simulink model "classic_dtc_winder_clean"  (R2026a)
settings: Solver=VariableStepAuto  StopTime=Tsim  MaxStep=1e-6
undefined symbols (not defined in the file): B, C_web, draw_max, draw_takeup, F0, F_ref, F_slack, ff_full, ff_on, filt_on, Fmax, h, H0, HB_lambda, HB_torque, Jc, Jm, K_web, Ki_F, Ki_speed, Kp_F, Kp_speed, lambda_ref, p, r0, rc, rho, rmax, Rs, Rs_factor, T_ramp, t_rev, tau_F, Tmax, Ts_dtc, v_line_set, Vdc, w, w_max, w_min, w_ref, web_w, winder_mode_set
libraries: nesl_utility x13, fl_lib x10, ee_lib x5, slpidlib x2
settings Model: Creator=kunal  LastModifiedBy=kunal
settings SimscapeCC: SimscapeLogType=none

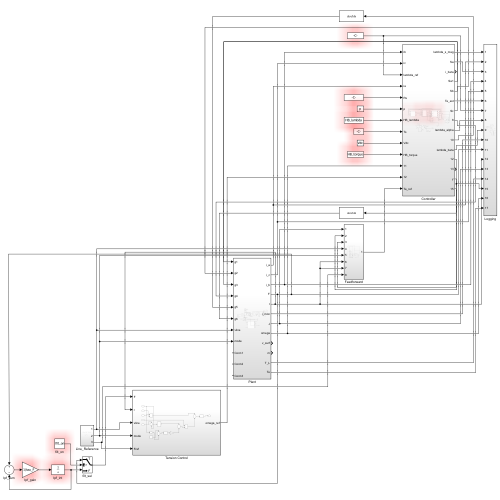
[thumbnail: Simulink's stored preview of the top-level diagram]
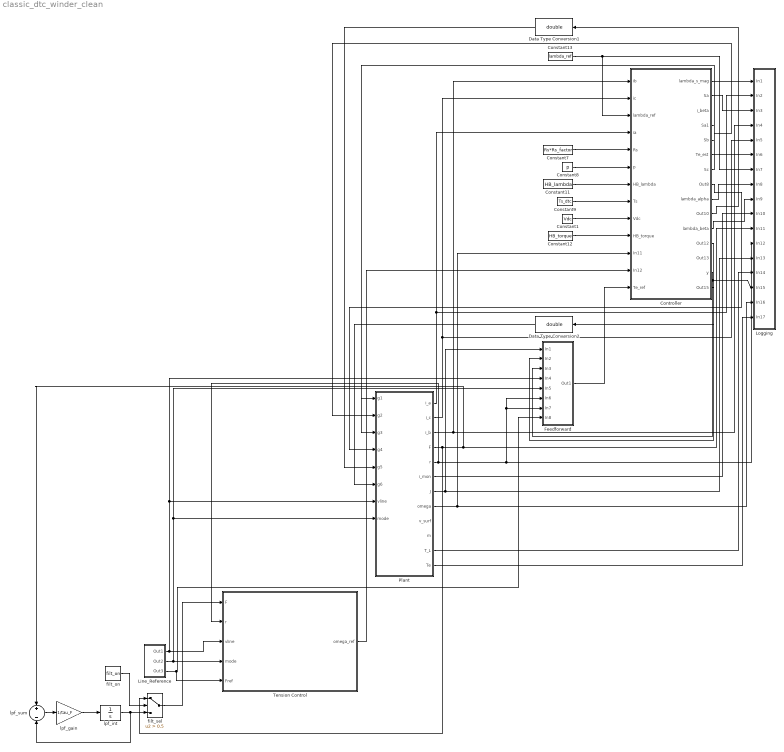
== system classic_dtc_winder_clean ==
  Constant1 : Constant  Value=Vdc
  Constant11 : Constant  Value=HB_lambda
  Constant12 : Constant  Value=HB_torque
  Constant13 : Constant  Value=lambda_ref
  Constant7 : Constant  Value=Rs*Rs_factor
  Constant8 : Constant  Value=p
  Constant9 : Constant  Value=Ts_dtc
  Controller : Subsystem
  Data Type Conversion1 : DataTypeConversion  OutDataTypeStr=double  SaturateOnIntegerOverflow=off  RndMeth=Floor
  Data Type Conversion2 : DataTypeConversion  OutDataTypeStr=double  SaturateOnIntegerOverflow=off  RndMeth=Floor
  Feedforward : Subsystem
  Line_Reference : Subsystem
  Logging : Subsystem
  Plant : Subsystem
  Tension Control : Subsystem
  filt_on : Constant  Value=filt_on
  filt_sel : Switch  Criteria=u2 > Threshold  Threshold=0.5  SaturateOnIntegerOverflow=off  InputSameDT=off
  lpf_gain : Gain  Gain=1/tau_F
  lpf_int : Integrator  InitialCondition=F0
  lpf_sum : Sum  Inputs=+-
  wires:
  lpf_sum/1 -> lpf_gain/1
  filt_on/1 -> filt_sel/2
  lpf_gain/1 -> lpf_int/1
  filt_sel/1 -> Tension Control/1(F)
  lpf_int/1 -> lpf_sum/2, filt_sel/3
  Line_Reference/3(Out3) -> Feedforward/8(In8), Tension Control/5(Fref)
  Line_Reference/1(Out1) -> Feedforward/4(In4), Plant/7(vline), Tension Control/3(vline)
  Line_Reference/2(Out2) -> Feedforward/5(In5), Plant/8(mode), Tension Control/4(mode)
  Plant/6(i_mon) -> Logging/10(In10)
  Plant/2(i_c) -> Logging/5(In5), Controller/2(ic)
  Tension Control/1(omega_ref) -> Controller/12(In12)
  Controller/1(lambda_s_mag) -> Logging/1(In1)
  Plant/1(i_a) -> Logging/2(In2), Controller/4(ia)
  Plant/11(T_L) -> Logging/14(In14)
  Plant/7(J) -> Logging/13(In13), Feedforward/1(In1)
  Plant/3(i_b) -> Controller/1(ib), Logging/4(In4)
  Plant/12(Te) -> Logging/17(In17)
  Plant/8(omega) -> Logging/16(In16), Controller/11(In11)
  Plant/4(F) -> lpf_sum/1, Logging/11(In11), filt_sel/1
  Plant/5(r) -> Feedforward/7(In7), Feedforward/6(In6), Logging/12(In12), Tension Control/2(r)
  Constant8/1 -> Controller/6(p)
  Data Type Conversion1/1 -> Plant/5(g5)
  Data Type Conversion2/1 -> Plant/6(g6)
  Constant11/1 -> Controller/7(HB_lambda)
  Constant13/1 -> Logging/7(In7), Controller/3(lambda_ref)
  Constant9/1 -> Controller/8(Ts)
  Constant7/1 -> Controller/5(Rs)
  Controller/11(lambda_beta) -> Logging/9(In9)
  Constant12/1 -> Controller/10(HB_torque)
  Constant1/1 -> Controller/9(Vdc)
  Feedforward/1(Out1) -> Controller/13(Te_ref)
  Controller/2(Sa) -> Logging/3(In3)
  Controller/4(Sa1) -> Plant/1(g1)
  Controller/5(Sb) -> Plant/2(g2)
  Controller/6(Te_est) -> Logging/6(In6)
  Controller/7(Sc) -> Plant/3(g3)
  Controller/8(Out8) -> Plant/4(g4)
  Controller/9(lambda_alpha) -> Logging/8(In8)
  Controller/10(Out10) -> Data Type Conversion1/1
  Controller/12(Out12) -> Data Type Conversion2/1
  Controller/14(y) -> Feedforward/3(In3), Logging/15(In15)
  Controller/15(Out15) -> Feedforward/2(In2)

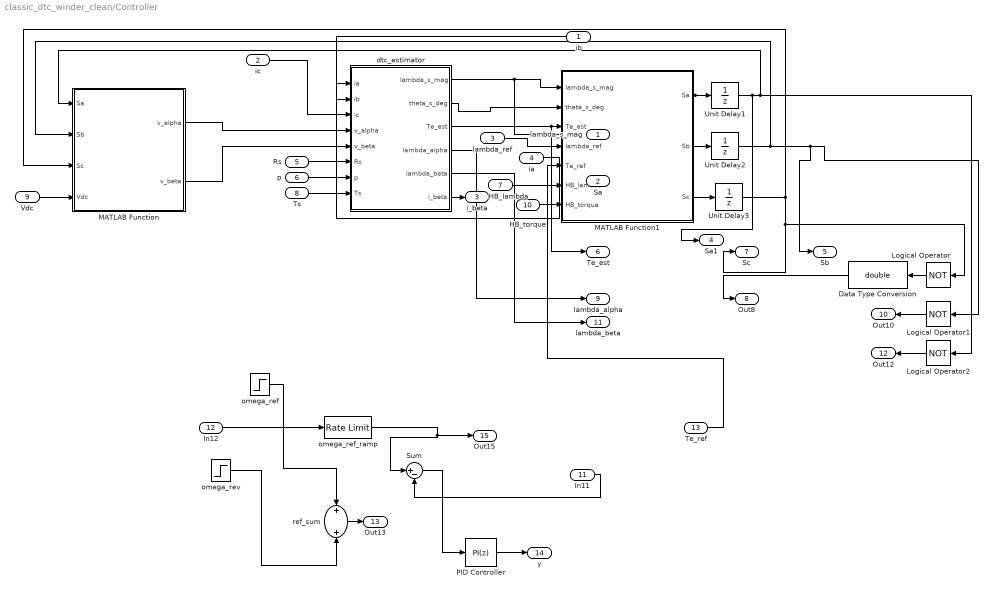
== system classic_dtc_winder_clean/Controller ==
  ib : Inport
  ic : Inport  Port=2
  lambda_ref : Inport  Port=3
  ia : Inport  Port=4
  Rs : Inport  Port=5
  p : Inport  Port=6
  HB_lambda : Inport  Port=7
  Ts : Inport  Port=8
  Vdc : Inport  Port=9
  HB_torque : Inport  Port=10
  In11 : Inport  Port=11
  In12 : Inport  Port=12
  Te_ref : Inport  Port=13
  Data Type Conversion : DataTypeConversion  OutDataTypeStr=double  SaturateOnIntegerOverflow=off  RndMeth=Floor
  Logical Operator : Logic  Operator=NOT  AllPortsSameDT=off  OutDataTypeStr=boolean
  Logical Operator1 : Logic  Operator=NOT  AllPortsSameDT=off  OutDataTypeStr=boolean
  Logical Operator2 : Logic  Operator=NOT  AllPortsSameDT=off  OutDataTypeStr=boolean
  MATLAB Function : MATLAB Function  TreatAsAtomicUnit=on  SystemSampleTime=Ts_dtc
  MATLAB Function1 : MATLAB Function  TreatAsAtomicUnit=on  SystemSampleTime=Ts_dtc
  PID Controller : slpidlib/PID Controller  Controller=PI  Form=Parallel  TimeDomain=Discrete-time  UseExternalTs=off  SampleTime=Ts_dtc  IntegratorMethod=Forward Euler  FilterMethod=Forward Euler  ControllerParametersSource=internal  P=Kp_speed  I=Ki_speed  UseKiTs=off  D=0  UseExternalDerivativeSource=off  N=100  UseFilter=on  TunerSelectOption=Transfer Function Based (PID Tuner App)  InitialConditionSource=internal  InitialConditionForIntegrator=0  InitialConditionForFilter=0  DifferentiatorICPrevScaledInput=0  ExternalReset=none  TrackingMode=off  Kt=1  LimitOutput=on  SatLimitsSource=internal  UpperSaturationLimit=5  LowerSaturationLimit=-5  LinearizeAsGain=on  AntiWindupMode=clamping  Kb=1  LimitIntegrator=off  UpperIntegratorSaturationLimit=inf  LowerIntegratorSaturationLimit=-inf  POutMin=[]  POutMax=[]  IOutMin=[]  IOutMax=[]  DOutMin=[]  DOutMax=[]  NOutMin=[]  NOutMax=[]  SumOutMin=[]  SumOutMax=[]  SaturationOutMin=[]  SaturationOutMax=[]  PParamMin=[]  PParamMax=[]  IParamMin=[]  IParamMax=[]  DParamMin=[]  DParamMax=[]  NParamMin=[]  NParamMax=[]  KbParamMin=[]  KbParamMax=[]  KtParamMin=[]  KtParamMax=[]  KbOutMin=[]  KbOutMax=[]  KtOutMin=[]  KtOutMax=[]  IntegratorOutMin=[]  IntegratorOutMax=[]  FilterOutMin=[]  FilterOutMax=[]  SumI1OutMin=[]  SumI1OutMax=[]  SumI2OutMin=[]  SumI2OutMax=[]  SumI3OutMin=[]  SumI3OutMax=[]  SumI4OutMin=[]  SumI4OutMax=[]  SumDOutMin=[]  SumDOutMax=[]  DifferentiatorOutMin=[]  DifferentiatorOutMax=[]  FilterDiffOutCoefMin=[]  FilterDiffOutCoefMax=[]  ReciprocalOutMin=[]  ReciprocalOutMax=[]  SumDenOutMin=[]  SumDenOutMax=[]  SumNumOutMin=[]  SumNumOutMax=[]  DivideOutMin=[]  DivideOutMax=[]  UdiffTsProdOutMin=[]  UdiffTsProdOutMax=[]  NTsProdOutMin=[]  NTsProdOutMax=[]  UintegralTsProdOutMin=[]  UintegralTsProdOutMax=[]  UngainTsProdOutMin=[]  UngainTsProdOutMax=[]  ClampingZeroOutDataTypeStr=Inherit: Inherit via back propagation  ClampingZeroOutMin=[]  ClampingZeroOutMax=[]  FilterDenConstantOutDataTypeStr=Inherit: Inherit via back propagation  FilterDenConstantOutMin=[]  FilterDenConstantOutMax=[]  PCopyOutDataTypeStr=Inherit: Inherit via back propagation  PCopyOutMin=[]  PCopyOutMax=[]  NCopyOutDataTypeStr=Inherit: Inherit via back propagation  NCopyOutMin=[]  NCopyOutMax=[]  IntegratorContinuousStateAttributes=''  IntegratorStateMustResolveToSignalObject=off  IntegratorRTWStateStorageClass=Auto  FilterContinuousStateAttributes=''  FilterStateMustResolveToSignalObject=off  FilterRTWStateStorageClass=Auto  ParallelPVariant=InternalParameters  IdealPVariant=Disabled  IVariant=InternalParameters  DVariant=Disabled  IntegratorVariant=Discrete  SatVariant=Enabled  AWVariant=DiscClampingParallel  PCopyVariant=Disabled  TRVariant=Disabled  FdbkBlocksVariant=Forward  IdealPFdbkVariant=Disabled  SatFdbkVariant=Disabled  DerivativeFilterVariant=Disabled  NVariant=Disabled  NCopyVariant=Disabled_SignalSpec  FilterICVariant=Disabled  IntegratorICVariant=InternalICs  ExternalResetVariant=Disabled  TRSumVariant=Passthrough  SumFdbkVariant=Disabled  SumVariant=Sum_PI  TsampFilterVariant=InternalTs  TsampNgainVariant=Passthrough  TsampIntegralVariant=Disabled_SignalSpec  ExternalSaturationOutDataTypeStr=Inherit: Same as second input  DerivativeSourceVariant=Disabled  PreIntVariant=InternalPreInt
  Sum : Sum  Inputs=|+-
  Unit Delay1 : UnitDelay  SampleTime=Ts_dtc
  Unit Delay2 : UnitDelay  SampleTime=Ts_dtc
  Unit Delay3 : UnitDelay  SampleTime=Ts_dtc
  dtc_estimator : MATLAB Function  TreatAsAtomicUnit=on  SystemSampleTime=Ts_dtc
  omega_ref : Step  Time=0.05  FinalValue=w_ref  SampleTime=Ts_dtc
  omega_ref_ramp : RateLimiter  RisingSlewLimit=700  FallingSlewLimit=-700  SampleTimeMode=inherited
  omega_rev : Step  Time=t_rev  FinalValue=-2*w_ref  SampleTime=Ts_dtc
  ref_sum : Sum
  lambda_s_mag : Outport
  Sa : Outport  Port=2
  i_beta : Outport  Port=3
  Sa1 : Outport  Port=4
  Sb : Outport  Port=5
  Te_est : Outport  Port=6
  Sc : Outport  Port=7
  Out8 : Outport  Port=8
  lambda_alpha : Outport  Port=9
  Out10 : Outport  Port=10
  lambda_beta : Outport  Port=11
  Out12 : Outport  Port=12
  Out13 : Outport  Port=13
  y : Outport  Port=14
  Out15 : Outport  Port=15
  wires:
  dtc_estimator/4(lambda_alpha) -> lambda_alpha/1
  Unit Delay1/1 -> Logical Operator2/1, MATLAB Function/1(Sa), Sa1/1
  omega_ref_ramp/1 -> Sum/1, Out15/1
  Logical Operator/1 -> Data Type Conversion/1
  MATLAB Function1/3(Sc) -> Unit Delay3/1
  Unit Delay3/1 -> Logical Operator/1, Sc/1, MATLAB Function/3(Sc)
  omega_ref/1 -> ref_sum/1
  omega_rev/1 -> ref_sum/2
  Vdc/1 -> MATLAB Function/4(Vdc)
  dtc_estimator/3(Te_est) -> Te_est/1, MATLAB Function1/3(Te_est)
  MATLAB Function/1(v_alpha) -> dtc_estimator/4(v_alpha)
  dtc_estimator/1(lambda_s_mag) -> lambda_s_mag/1, MATLAB Function1/1(lambda_s_mag)
  MATLAB Function1/1(Sa) -> Unit Delay1/1, Sa/1
  In11/1 -> Sum/2
  ref_sum/1 -> Out13/1
  lambda_ref/1 -> MATLAB Function1/4(lambda_ref)
  MATLAB Function1/2(Sb) -> Unit Delay2/1
  dtc_estimator/6(i_beta) -> i_beta/1
  dtc_estimator/2(theta_s_deg) -> MATLAB Function1/2(theta_s_deg)
  Unit Delay2/1 -> Sb/1, Logical Operator1/1, MATLAB Function/2(Sb)
  Sum/1 -> PID Controller/1
  MATLAB Function/2(v_beta) -> dtc_estimator/5(v_beta)
  Te_ref/1 -> MATLAB Function1/5(Te_ref)
  Logical Operator1/1 -> Out10/1
  HB_lambda/1 -> MATLAB Function1/6(HB_lambda)
  Data Type Conversion/1 -> Out8/1
  In12/1 -> omega_ref_ramp/1
  Rs/1 -> dtc_estimator/6(Rs)
  ia/1 -> dtc_estimator/1(ia)
  HB_torque/1 -> MATLAB Function1/7(HB_torque)
  dtc_estimator/5(lambda_beta) -> lambda_beta/1
  Logical Operator2/1 -> Out12/1
  ic/1 -> dtc_estimator/3(ic)
  ib/1 -> dtc_estimator/2(ib)
  Ts/1 -> dtc_estimator/8(Ts)
  p/1 -> dtc_estimator/7(p)
  PID Controller/1 -> y/1

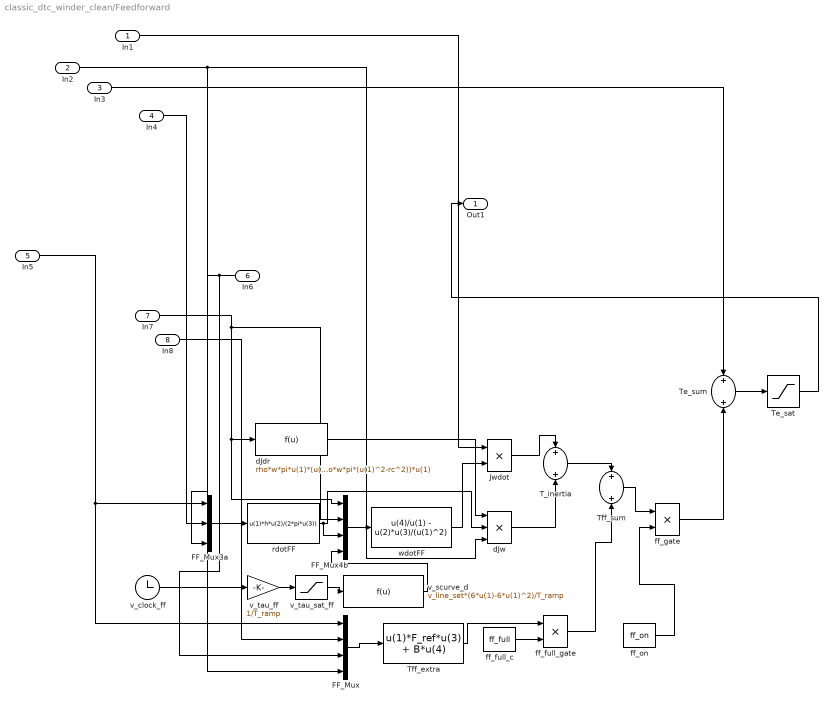
== system classic_dtc_winder_clean/Feedforward ==
  In1 : Inport
  In2 : Inport  Port=2
  In3 : Inport  Port=3
  In4 : Inport  Port=4
  In5 : Inport  Port=5
  In6 : Inport  Port=6
  In7 : Inport  Port=7
  In8 : Inport  Port=8
  FF_Mux : Mux
  FF_Mux3a : Mux  Inputs=3
  FF_Mux4b : Mux
  Jwdot : Product
  T_inertia : Sum
  Te_sat : Saturate  UpperLimit=Tmax  LowerLimit=-Tmax
  Te_sum : Sum
  Tff_extra : Fcn  Expr=u(1)*F_ref*u(3) + B*u(4)
  Tff_sum : Sum
  dJdr : Fcn  Expr=rho*w*pi*u(1)*(u(1)^2+rc^2) + (rho*w*pi*(u(1)^2-rc^2))*u(1)
  dJw : Product  Inputs=3
  ff_full_c : Constant  Value=ff_full
  ff_full_gate : Product
  ff_gate : Product
  ff_on : Constant  Value=ff_on
  rdotFF : Fcn  Expr=u(1)*h*u(2)/(2*pi*u(3))
  v_clock_ff : Clock
  v_scurve_d : Fcn  Expr=v_line_set*(6*u(1)-6*u(1)^2)/T_ramp
  v_tau_ff : Gain  Gain=1/T_ramp
  v_tau_sat_ff : Saturate  UpperLimit=1  LowerLimit=0
  wdotFF : Fcn  Expr=u(4)/u(1) - u(2)*u(3)/(u(1)^2)
  Out1 : Outport
  wires:
  Jwdot/1 -> T_inertia/1
  In3/1 -> Te_sum/1
  ff_gate/1 -> Te_sum/2
  FF_Mux3a/1 -> rdotFF/1
  In6/1 -> FF_Mux3a/3, FF_Mux/3
  v_tau_ff/1 -> v_tau_sat_ff/1
  ff_full_c/1 -> ff_full_gate/2
  In2/1 -> dJw/3, FF_Mux/4
  dJw/1 -> T_inertia/2
  In5/1 -> FF_Mux3a/1, FF_Mux/1
  ff_on/1 -> ff_gate/2
  dJdr/1 -> dJw/1
  In8/1 -> FF_Mux/2
  Te_sum/1 -> Te_sat/1
  v_tau_sat_ff/1 -> v_scurve_d/1
  v_scurve_d/1 -> FF_Mux4b/4
  rdotFF/1 -> FF_Mux4b/3, dJw/2
  v_clock_ff/1 -> v_tau_ff/1
  FF_Mux/1 -> Tff_extra/1
  FF_Mux4b/1 -> wdotFF/1
  Tff_extra/1 -> ff_full_gate/1
  Te_sat/1 -> Out1/1
  wdotFF/1 -> Jwdot/2
  T_inertia/1 -> Tff_sum/1
  ff_full_gate/1 -> Tff_sum/2
  Tff_sum/1 -> ff_gate/1
  In7/1 -> FF_Mux4b/2, dJdr/1, FF_Mux4b/1
  In1/1 -> Jwdot/1
  In4/1 -> FF_Mux3a/2

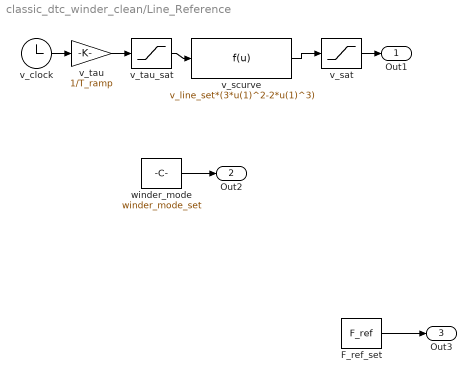
== system classic_dtc_winder_clean/Line_Reference ==
  F_ref_set : Constant  Value=F_ref
  v_clock : Clock
  v_sat : Saturate  UpperLimit=v_line_set  LowerLimit=0
  v_scurve : Fcn  Expr=v_line_set*(3*u(1)^2-2*u(1)^3)
  v_tau : Gain  Gain=1/T_ramp
  v_tau_sat : Saturate  UpperLimit=1  LowerLimit=0
  winder_mode : Constant  Value=winder_mode_set
  Out1 : Outport
  Out2 : Outport  Port=2
  Out3 : Outport  Port=3
  wires:
  v_sat/1 -> Out1/1
  F_ref_set/1 -> Out3/1
  v_tau/1 -> v_tau_sat/1
  winder_mode/1 -> Out2/1
  v_tau_sat/1 -> v_scurve/1
  v_clock/1 -> v_tau/1
  v_scurve/1 -> v_sat/1

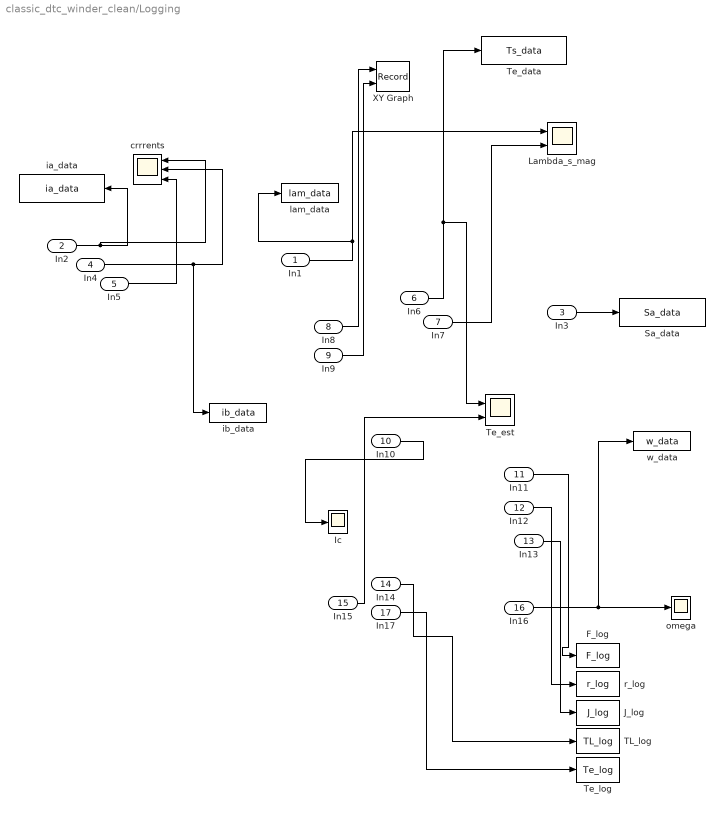
== system classic_dtc_winder_clean/Logging ==
  In1 : Inport
  In2 : Inport  Port=2
  In3 : Inport  Port=3
  In4 : Inport  Port=4
  In5 : Inport  Port=5
  In6 : Inport  Port=6
  In7 : Inport  Port=7
  In8 : Inport  Port=8
  In9 : Inport  Port=9
  In10 : Inport  Port=10
  In11 : Inport  Port=11
  In12 : Inport  Port=12
  In13 : Inport  Port=13
  In14 : Inport  Port=14
  In15 : Inport  Port=15
  In16 : Inport  Port=16
  In17 : Inport  Port=17
  F_log : ToWorkspace  VariableName=F_log  SaveFormat=Timeseries  SampleTime=-1
  Ic : Scope
      settings: ActiveDisplayYMinimum=-1.574268599657235  ActiveDisplayYMaximum=1.0954007787431075  DataLoggingVariableName=ScopeData3
  J_log : ToWorkspace  VariableName=J_log  SaveFormat=Timeseries  SampleTime=-1
  Lambda_s_mag : Scope  NumInputPorts=2
      settings: ActiveDisplayYMinimum=0.17238629365269534  ActiveDisplayYMaximum=0.17761260298821638
  Sa_data : ToWorkspace  VariableName=Sa_data  SaveFormat=Timeseries  SampleTime=-1
  TL_log : ToWorkspace  VariableName=TL_log  SaveFormat=Timeseries  SampleTime=-1
  Te_data : ToWorkspace  VariableName=Ts_data  SaveFormat=Timeseries  SampleTime=-1
  Te_est : Scope  NumInputPorts=2
      settings: ActiveDisplayYMinimum=-0.7454839045495818  ActiveDisplayYMaximum=5.7226303419643028
  Te_log : ToWorkspace  VariableName=Te_log  SaveFormat=Timeseries  SampleTime=-1
  XY Graph : Record  NumPorts=2.0  FileSettingsInternal="{\"entries\":[{\"content\":{\"excelSettings\":{\"content\":{},\"type\":\"Streamout.ExcelSettings\"},\"parquetSettings\":{\"content\":{},\"type\":\"Streamout.ParquetSettings\"}},\"type\":\"Streamout.FileSettingStorage\",\"uuid\":\"\"}],\"packageUris\":[\"http:\\/\\/schema.mathworks.com\\/mf0\\/streamout_blocks\\/R2020a\"],\"version\":\"1.0\"}"  FrameSettings=[0, 0]  Layout=[1 1]  SignalsInternal="{\"entries\":[{\"content\":{\"signals\":[{\"content\":{\"blockPath\":[],\"dimensions\":[1],\"domain\":\"\",\"lineColor\":\"#edb120\",\"lineWidth\":2,\"port\":1,\"signalID\":1},\"type\":\"RecordBlkView.Signal\",\"uuid\":\"\"},{\"content\":{\"blockPath\":[],\"dimensions\":[1],\"domain\":\"\",\"lineColor\":\"#a2142f\",\"lineWidth\":2,\"plots\":[ 1 ],\"port\":1,\"signalID\":2,\"signalName\":\"dtc_estimator:4\"},\"type\":\"RecordBlkView.Signal\",\"uuid\":\"\"},{\"content\":{\"blockPath\":[],\"dimensions\":[1],\"domain\":\"\",\"lineColor\":\"#4dbeee\",\"lineWidth\":2,\"port\":1,\"signalID\":3,\"signalName\":\"MATLAB Function1:1\"},\"type\":\"RecordBlkView.Signal\",\"uuid\":\"\"},{\"content\":{\"blockPath\":[],\"dimensions\":[1],\"domain\":\"\",\"lineColor\":\"#a2142f\",\"lineWidth\":2,\"port\":1,\"signalID\":4,\"signalName\":\"dtc_estimator:3\"},\"type\":\"RecordBlkView.Signal\",\"uuid\":\"\"},{\"content\":{\"blockPath\":[],\"dimensions\":[1],\"domain\":\"\",\"lineColor\":\"#139fff\",\"lineWidth\":2,\"port\":1,\"signalID\":5,\"signalName\":\"PS-Simulink\\nConverter6\"},\"type\":\"RecordBlkView.Signal\",\"uuid\":\"\"},{\"content\":{\"blockPath\":[],\"dimensions\":[1],\"domain\":\"\",\"lineColor\":\"#139fff\",\"lineWidth\":2,\"plots\":[ 1 ],\"port\":2,\"signalID\":6,\"signalName\":\"dtc_estimator:5\"},\"type\":\"RecordBlkView.Signal\",\"uuid\":\"\"}]},\"type\":\"RecordBlkView.InputSignals\",\"uuid\":\"\"}],\"packageUris\":[\"http:\\/\\/schema.mathworks.com\\/mf0\\/streamout_blocks\\/R2020a\"],\"version\":\"1.0\"}"  VisualizationBindings="{\"xyplotplugin\":{\"info\":[{\"series\":[{\"bindingParametersList\":[{\"parameter\":\"X-Axis\",\"signalID\":6,\"signalName\":\"dtc_estimator:5\"},{\"parameter\":\"Y-Axis\",\"signalID\":2,\"signalName\":\"dtc_estimator:4\"}],\"seriesID\":0}],\"subplotID\":1}]}}"  CompatibilityTag=XY
  crrrents : Scope  NumInputPorts=3
      settings: ActiveDisplayYMinimum=-0.84095457498460979  ActiveDisplayYMaximum=0.85331725762283572  DataLoggingVariableName=ScopeData13
  ia_data : ToWorkspace  VariableName=ia_data  SaveFormat=Timeseries  SampleTime=-1
  ib_data : ToWorkspace  VariableName=ib_data  SaveFormat=Timeseries  SampleTime=-1
  lam_data : ToWorkspace  VariableName=lam_data  SaveFormat=Timeseries  SampleTime=-1
  omega : Scope
      settings: ActiveDisplayYMinimum=4.4842627024722095  ActiveDisplayYMaximum=29.582290486365775  DataLoggingVariableName=ScopeData2
  r_log : ToWorkspace  VariableName=r_log  SaveFormat=Timeseries  SampleTime=-1
  w_data : ToWorkspace  VariableName=w_data  SaveFormat=Timeseries  SampleTime=-1
  wires:
  In17/1 -> Te_log/1
  In10/1 -> Ic/1
  In8/1 -> XY Graph/1
  In4/1 -> crrrents/2, ib_data/1
  In9/1 -> XY Graph/2
  In14/1 -> TL_log/1
  In16/1 -> omega/1, w_data/1
  In2/1 -> crrrents/1, ia_data/1
  In6/1 -> Te_data/1, Te_est/1
  In1/1 -> Lambda_s_mag/1, lam_data/1
  In3/1 -> Sa_data/1
  In11/1 -> F_log/1
  In13/1 -> J_log/1
  In15/1 -> Te_est/2
  In12/1 -> r_log/1
  In7/1 -> Lambda_s_mag/2
  In5/1 -> crrrents/3

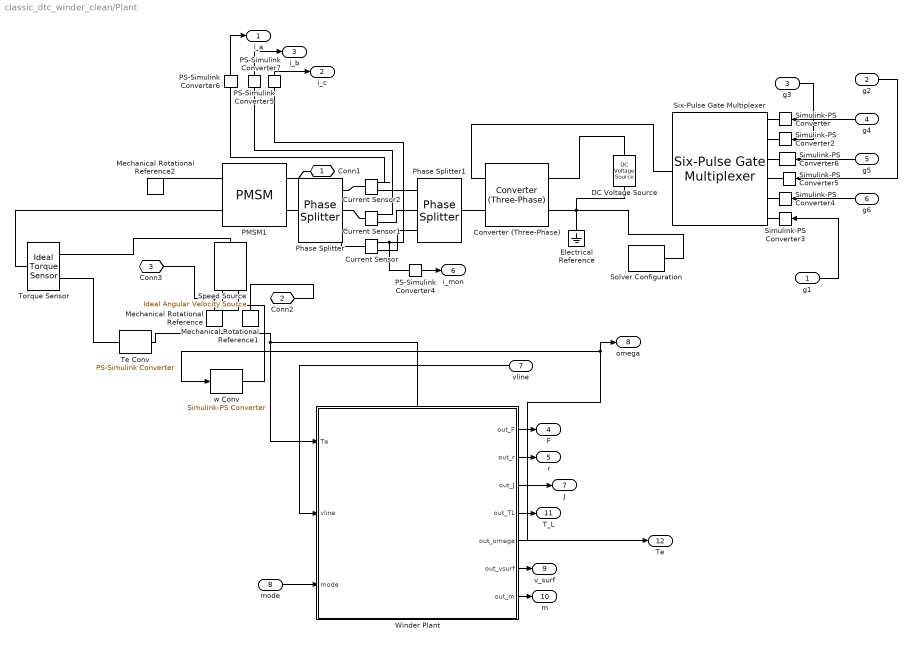
== system classic_dtc_winder_clean/Plant ==
  g1 : Inport
  g2 : Inport  Port=2
  g3 : Inport  Port=3
  g4 : Inport  Port=4
  g5 : Inport  Port=5
  g6 : Inport  Port=6
  vline : Inport  Port=7
  mode : Inport  Port=8
  Converter (Three-Phase) : ee_lib/Semiconductors & Converters/Converters/Converter (Three-Phase)  port_option=ee.enum.threePhasePort.composite  fidelity_option=ee.enum.converters.fidelity.detailed  device_type=ee.enum.converters.switchingdevice.ideal  showThermalPort=false  K=0  Vth=0.5 V  Vgt=1 V  Vgt_off=-1 V  Ih=1 A  Vf=0.8 V  Ron=0.001 Ohm  Rds=0.001 Ohm  Goff=1e-6 1/Ohm  Eon_scalar=22.86e-3 J  Eoff_scalar=17.14e-3 J  Eoff_natural_commutation=10e-3 J  Voff=300 V  Iout_scalar=600 A  onCurrentMeasDelay=0 s  useCurrentFromPreviousCycle=false  useVoltageFromPreviousCycle=false  diode_param=ee.enum.converters.protectiondiode.nodynamics  diode_Vf=0.8 V  diode_Ron=0.001 Ohm  diode_Goff=1e-5 1/Ohm  diode_C=50 nF  diode_iRM=-235 A  diode_iF=300 A  diode_idot=-50 A/us  diode_trr_param=ee.enum.converters.diodetrr.trr_factor  diode_trr_factor=3  diode_trr=15 us  diode_Qrr=1500 s*uA  diode_rec_loss_model=ee.enum.diode.reverseRecoveryModel.fixed  diode_ErecVal=0 J  diode_scaleWithIandV=false  diode_ErecMat=zeros(2, 3) J  diode_TjrecVec=[298.15, 398.15] K  diode_IfrecVec=[.1, 1, 10] A  diode_IrecVal=10 A  diode_VrecVal=10 V  diode_tFilter=1 / 1000 / 100 s  thermal_network_parameterization=ee.enum.thermalNetworkTopology.external  Rth=[.08, .5] K/W  Rth_Cauer=[.08, .1, .5] K/W  Rth_Foster=[.08, .14, .22, .16] K/W  thermal_mass_parameterization=ee.enum.thermalNetwork.timeconstant  thermal_mass=[.01, .5] J/K  thermal_mass_Cauer=[.01, .1, .5] J/K  thermal_mass_Foster=[.001, .005, .05, .5] J/K  thermal_time_constant=[.001, .2] s  thermal_time_constant_Cauer=[.001, .1, .2] s  thermal_time_constant_Foster=[7e-05, .0007, .01, .08] s  thermal_mass_initial_temperatures=[25, 25] degC  thermal_mass_initial_temperatures_Cauer=[25, 25, 25] degC  junction_thermal_mass=0.01 J/K  Tvec_initial_Foster=[25, 25, 25, 25] degC  snubber_type=ee.enum.converters.snubber.exclude  Cs=1e-7 F  Rs=0.1 Ohm  Vce_loss=[0, 150, 300] V
  Current Sensor : fl_lib/Electrical/Electrical Sensors/Current Sensor
  Current Sensor1 : fl_lib/Electrical/Electrical Sensors/Current Sensor
  Current Sensor2 : fl_lib/Electrical/Electrical Sensors/Current Sensor
  DC Voltage Source : fl_lib/Electrical/Electrical Sources/DC Voltage Source  v0=Vdc V
  Electrical Reference : fl_lib/Electrical/Electrical Elements/Electrical Reference
  Mechanical Rotational Reference : fl_lib/Mechanical/Rotational Elements/Mechanical Rotational Reference
  Mechanical Rotational Reference1 : fl_lib/Mechanical/Rotational Elements/Mechanical Rotational Reference
  Mechanical Rotational Reference2 : fl_lib/Mechanical/Rotational Elements/Mechanical Rotational Reference
  PMSM1 : ee_lib/Electromechanical/Permanent Magnet/PMSM  port_option=ee.enum.threePhasePort.composite  winding_type=ee.enum.electromech.statorconfiguration.wye  machine_param=ee.enum.pmsm.parameterization.constant  nPolePairs=p  pmflux_param=ee.enum.pmflux.fluxlinkage  pm_flux_linkage=lambda_f Wb  torque_constant=0.18 N*m/A  back_emf_constant=0.18 V*s/rad  stator_param=ee.enum.statorparam.LdLqL0  Ld=Ld H  Lq=Lq H  idVec=[-200, 0, 200] A  iqVec=[-200, 0, 200] A  LdMatrix=0.0002 * ones(3, 3) H  LqMatrix=0.0002 * ones(3, 3) H  PmMatrix=0.1 * ones(3, 3) Wb  ktMatrix=0.18 * ones(3, 3) N*m/A  keMatrix=0.18 * ones(3, 3) V*s/rad  L0=0.00016 H  Ls=0.0002 H  Lm=-0.00002 H  Ms=0.00002 H  Rs=Rs Ohm  zero_sequence=ee.enum.park.zerosequence.include  axes_param=ee.enum.rotorangle.daxis  loss_param=ee.enum.ironloss.none  losses_oc=[0, 0, 0] W  losses_sc=[0, 0, 0] W  f_losses=60 Hz  Isc_losses=95 A  J=0 kg*m^2  lam=0 N*m*s/rad  i_d_specify=off  i_d_priority=None  i_d=0 A  i_d_nominal_specify=off  i_d_nominal_value=1  i_d_nominal_unit=A  i_q_specify=off  i_q_priority=None  i_q=0 A  i_q_nominal_specify=off  i_q_nominal_value=1  i_q_nominal_unit=A  torque_specify=off  torque_priority=None  torque=0 N*m  torque_nominal_specify=off  torque_nominal_value=1  torque_nominal_unit=N*m  angular_velocity_specify=off  angular_velocity_priority=High  angular_velocity=0 rpm  angular_velocity_nominal_specify=off  angular_velocity_nominal_value=1  angular_velocity_nominal_unit=rpm  angular_position_specify=off  angular_position_priority=High  angular_position=0 deg  angular_position_nominal_specify=off  angular_position_nominal_value=1  angular_position_nominal_unit=deg  alpha=3.93e-3 1/K  alpha_flux=-0.001 1/K  Tmeas=298.15 K  stator_thermal_mass=100 J/K  rotor_thermal_mass=200 J/K  Rm_percent_rotor=90  Rd_percent_rotor=30  temperatureA_specify=off  temperatureA_priority=High  temperatureA=25 degC  temperatureA_nominal_specify=off  temperatureA_nominal_value=1  temperatureA_nominal_unit=degC  temperatureB_specify=off  temperatureB_priority=High  temperatureB=25 degC  temperatureB_nominal_specify=off  temperatureB_nominal_value=1  temperatureB_nominal_unit=degC  temperatureC_specify=off  temperatureC_priority=High  temperatureC=25 degC  temperatureC_nominal_specify=off  temperatureC_nominal_value=1  temperatureC_nominal_unit=degC  temperatureR_specify=off  temperatureR_priority=High  temperatureR=25 degC  temperatureR_nominal_specify=off  temperatureR_nominal_value=1  temperatureR_nominal_unit=degC
  PS-Simulink Converter{4..7} (4 alike) : nesl_utility/PS-Simulink Converter  PhysicalDomain=network_engine_domain  SubClassName=ps_output  LeftPortType=input  RightPortType=output  PseudoPeriodic=off  Frequencies=[]  VectorFormat=inherit  Unit=inherit  AffineConversion=off
  Phase Splitter : ee_lib/Connectors & References/Phase Splitter
  Phase Splitter1 : ee_lib/Connectors & References/Phase Splitter
  Simulink-PS Converter{,2..6} (6 alike) : nesl_utility/Simulink-PS Converter  PhysicalDomain=network_engine_domain  SubClassName=ps_input  LeftPortType=input  RightPortType=output  PseudoPeriodic=off  Frequencies=[]  NoiseDistribution=none  NoiseParameters=[]  Unit=1  AffineConversion=off  FilteringAndDerivatives=provide  SimscapeFilterOrder=1  InputFilterTimeConstant=0.001  UdotUserProvided=0
  Six-Pulse Gate Multiplexer : ee_lib/Semiconductors & Converters/Converters/Six-Pulse Gate Multiplexer  port_option=ee.enum.controlport.ps
  Solver Configuration : nesl_utility/Solver Configuration  PhysicalDomain=network_engine_domain  SubClassName=solver  LeftPortType=input  RightPortType=generic  Tones=[]  Harmonics=[]  SimulateNoise=off  Profile=off  UseLocalSampling=off  EnableSwitchedLinearOptims=on  FrequencyDomain=off  UseCCode=off  RelTol=0.001  AbsTol=0.001  MinStep=1e-09  ToWorkspace=off  RevertToSquareIcSolve=off  NumHomotopyIterations=100  PhasorMode=off  PhasorModeNumHarmonics=1  ConsistencySolver=NEWTON_XTOL_AFTER_FTOL  CanonicalOrdering=CANONICAL  OptimizeIntermediates=OPTIMIZED  IndexReductionMethod=DerivativeReplacement  DoDC=off  ResidualTolerance=1e-09  ConsistencyTolSource=GLOBAL  ConsistencyAbsTol=0.001  ConsistencyRelTol=0.001  ConsistencyTolFactor=0.001  UseLocalSolver=off  LocalSolverChoice=NE_BACKWARD_EULER_ADVANCER  ResolveIndetEquations=on  FunctionEvalNumThread=1  LocalSolverSampleTime=0.001  DoFixedCost=off  MaxNonlinIter=3  MaxModeIter=2  ComputeImpulses=off  ImpulseIterations=2  LinearAlgebra=auto  LinearAlgebraNumThread=0  EquationFormulation=NE_TIME_EF  DelaysMemoryBudget=1024  AutomaticFiltering=on  FilteringTimeConstant=0.001  PartitionStorageMethod=AS_NEEDED  PartitionMemoryBudget=1024  PartitionMethod=ROBUST  MultibodyUseLocalSolver=off  MultibodyLocalSolverChoice=ODE1  MultibodyLocalSolverSampleTime=0.001
  Speed Source : fl_lib/Mechanical/Mechanical Sources/Ideal Angular Velocity Source
  Te Conv : nesl_utility/PS-Simulink Converter  PhysicalDomain=network_engine_domain  SubClassName=ps_output  LeftPortType=input  RightPortType=output  PseudoPeriodic=off  Frequencies=[]  VectorFormat=inherit  Unit=inherit  AffineConversion=off
  Torque Sensor : fl_lib/Mechanical/Mechanical Sensors/Ideal Torque Sensor
  Winder Plant : Subsystem
  w Conv : nesl_utility/Simulink-PS Converter  PhysicalDomain=network_engine_domain  SubClassName=ps_input  LeftPortType=input  RightPortType=output  PseudoPeriodic=off  Frequencies=[]  NoiseDistribution=none  NoiseParameters=[]  Unit=1  AffineConversion=off  FilteringAndDerivatives=provide  SimscapeFilterOrder=1  InputFilterTimeConstant=0.001  UdotUserProvided=0
  Conn1 : PMIOPort  Side=Left
  Conn2 : PMIOPort  Port=2  Side=Left
  Conn3 : PMIOPort  Port=3  Side=Left
  i_a : Outport
  i_c : Outport  Port=2
  i_b : Outport  Port=3
  F : Outport  Port=4
  r : Outport  Port=5
  i_mon : Outport  Port=6
  J : Outport  Port=7
  omega : Outport  Port=8
  v_surf : Outport  Port=9
  m : Outport  Port=10
  T_L : Outport  Port=11
  Te : Outport  Port=12
  wires:
  g1/1 -> Simulink-PS Converter3/1
  Winder Plant/3(out_J) -> J/1
  g2/1 -> Simulink-PS Converter5/1
  g4/1 -> Simulink-PS Converter/1
  Winder Plant/2(out_r) -> r/1
  PS-Simulink Converter7/1 -> i_c/1
  Winder Plant/7(out_m) -> m/1
  g3/1 -> Simulink-PS Converter2/1
  g6/1 -> Simulink-PS Converter4/1
  PS-Simulink Converter5/1 -> i_b/1
  Winder Plant/4(out_TL) -> T_L/1
  Te Conv/1 -> Te/1, Winder Plant/1(Te)
  PS-Simulink Converter6/1 -> i_a/1
  mode/1 -> Winder Plant/3(mode)
  g5/1 -> Simulink-PS Converter6/1
  Winder Plant/5(out_omega) -> omega/1, w Conv/1
  vline/1 -> Winder Plant/2(vline)
  PS-Simulink Converter4/1 -> i_mon/1
  Winder Plant/6(out_vsurf) -> v_surf/1
  Winder Plant/1(out_F) -> F/1
  connections:
  PMSM1/RConn2 -- Mechanical Rotational Reference2/LConn1
  Current Sensor1/RConn1 -- PS-Simulink Converter5/LConn1
  PMSM1/RConn1 -- Torque Sensor/LConn1
  Electrical Reference/LConn1 -- Solver Configuration/RConn1 -- Converter (Three-Phase)/RConn2 -- DC Voltage Source/RConn1
  Current Sensor2/LConn1 -- Phase Splitter/RConn1
  Mechanical Rotational Reference/LConn1 -- Conn3/RConn1 -- Speed Source/RConn2
  Current Sensor/RConn1 -- PS-Simulink Converter7/LConn1 -- PS-Simulink Converter4/LConn1
  Six-Pulse Gate Multiplexer/RConn1 -- Converter (Three-Phase)/LConn1
  Current Sensor2/RConn1 -- PS-Simulink Converter6/LConn1
  Converter (Three-Phase)/LConn2 -- Phase Splitter1/LConn1
  Phase Splitter/RConn2 -- Current Sensor1/LConn1
  Torque Sensor/RConn1 -- Speed Source/LConn1
  Converter (Three-Phase)/RConn1 -- DC Voltage Source/LConn1
  PMSM1/LConn1 -- Phase Splitter/LConn1
  Phase Splitter1/RConn2 -- Current Sensor1/RConn2
  Simulink-PS Converter3/RConn1 -- Six-Pulse Gate Multiplexer/LConn1
  Current Sensor2/RConn2 -- Phase Splitter1/RConn1
  Phase Splitter/RConn3 -- Current Sensor/LConn1
  Simulink-PS Converter/RConn1 -- Six-Pulse Gate Multiplexer/LConn6
  Phase Splitter1/RConn3 -- Current Sensor/RConn2
  Simulink-PS Converter2/RConn1 -- Six-Pulse Gate Multiplexer/LConn5
  w Conv/RConn1 -- Speed Source/RConn1
  Simulink-PS Converter4/RConn1 -- Six-Pulse Gate Multiplexer/LConn2
  PMSM1/LConn2 -- Conn1/RConn1
  Simulink-PS Converter5/RConn1 -- Six-Pulse Gate Multiplexer/LConn3
  Simulink-PS Converter6/RConn1 -- Six-Pulse Gate Multiplexer/LConn4
  Torque Sensor/RConn2 -- Te Conv/LConn1
  Conn2/RConn1 -- Mechanical Rotational Reference1/LConn1

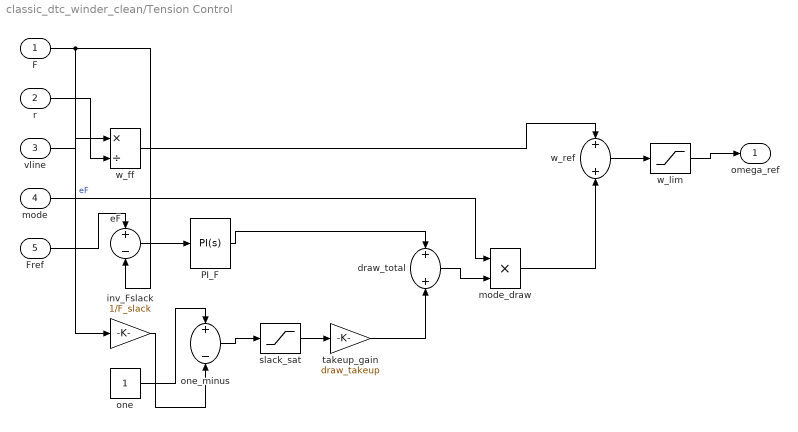
== system classic_dtc_winder_clean/Tension Control ==
  F : Inport
  r : Inport  Port=2
  vline : Inport  Port=3
  mode : Inport  Port=4
  Fref : Inport  Port=5
  PI_F : slpidlib/PID Controller  Controller=PI  Form=Parallel  TimeDomain=Continuous-time  UseExternalTs=off  SampleTime=-1  IntegratorMethod=Forward Euler  FilterMethod=Forward Euler  ControllerParametersSource=internal  P=Kp_F  I=Ki_F  UseKiTs=off  D=0  UseExternalDerivativeSource=off  N=100  UseFilter=on  TunerSelectOption=Transfer Function Based (PID Tuner App)  InitialConditionSource=internal  InitialConditionForIntegrator=0  InitialConditionForFilter=0  DifferentiatorICPrevScaledInput=0  ExternalReset=none  TrackingMode=off  Kt=1  LimitOutput=on  SatLimitsSource=internal  UpperSaturationLimit=draw_max  LowerSaturationLimit=-draw_max  LinearizeAsGain=on  AntiWindupMode=clamping  Kb=1  LimitIntegrator=off  UpperIntegratorSaturationLimit=inf  LowerIntegratorSaturationLimit=-inf  POutMin=[]  POutMax=[]  IOutMin=[]  IOutMax=[]  DOutMin=[]  DOutMax=[]  NOutMin=[]  NOutMax=[]  SumOutMin=[]  SumOutMax=[]  SaturationOutMin=[]  SaturationOutMax=[]  PParamMin=[]  PParamMax=[]  IParamMin=[]  IParamMax=[]  DParamMin=[]  DParamMax=[]  NParamMin=[]  NParamMax=[]  KbParamMin=[]  KbParamMax=[]  KtParamMin=[]  KtParamMax=[]  KbOutMin=[]  KbOutMax=[]  KtOutMin=[]  KtOutMax=[]  IntegratorOutMin=[]  IntegratorOutMax=[]  FilterOutMin=[]  FilterOutMax=[]  SumI1OutMin=[]  SumI1OutMax=[]  SumI2OutMin=[]  SumI2OutMax=[]  SumI3OutMin=[]  SumI3OutMax=[]  SumI4OutMin=[]  SumI4OutMax=[]  SumDOutMin=[]  SumDOutMax=[]  DifferentiatorOutMin=[]  DifferentiatorOutMax=[]  FilterDiffOutCoefMin=[]  FilterDiffOutCoefMax=[]  ReciprocalOutMin=[]  ReciprocalOutMax=[]  SumDenOutMin=[]  SumDenOutMax=[]  SumNumOutMin=[]  SumNumOutMax=[]  DivideOutMin=[]  DivideOutMax=[]  UdiffTsProdOutMin=[]  UdiffTsProdOutMax=[]  NTsProdOutMin=[]  NTsProdOutMax=[]  UintegralTsProdOutMin=[]  UintegralTsProdOutMax=[]  UngainTsProdOutMin=[]  UngainTsProdOutMax=[]  ClampingZeroOutDataTypeStr=Inherit: Inherit via back propagation  ClampingZeroOutMin=[]  ClampingZeroOutMax=[]  FilterDenConstantOutDataTypeStr=Inherit: Inherit via back propagation  FilterDenConstantOutMin=[]  FilterDenConstantOutMax=[]  PCopyOutDataTypeStr=Inherit: Inherit via back propagation  PCopyOutMin=[]  PCopyOutMax=[]  NCopyOutDataTypeStr=Inherit: Inherit via back propagation  NCopyOutMin=[]  NCopyOutMax=[]  IntegratorContinuousStateAttributes=''  IntegratorStateMustResolveToSignalObject=off  IntegratorRTWStateStorageClass=Auto  FilterContinuousStateAttributes=''  FilterStateMustResolveToSignalObject=off  FilterRTWStateStorageClass=Auto  ParallelPVariant=InternalParameters  IdealPVariant=Disabled  IVariant=InternalParameters  DVariant=Disabled  IntegratorVariant=Continuous  SatVariant=Enabled  AWVariant=ContClampingParallel  PCopyVariant=Disabled  TRVariant=Disabled  FdbkBlocksVariant=Forward  IdealPFdbkVariant=Disabled  SatFdbkVariant=Disabled  DerivativeFilterVariant=Disabled  NVariant=Disabled  NCopyVariant=Disabled_SignalSpec  FilterICVariant=Disabled  IntegratorICVariant=InternalICs  ExternalResetVariant=Disabled  TRSumVariant=Passthrough  SumFdbkVariant=Disabled  SumVariant=Sum_PI  TsampFilterVariant=InternalTs  TsampNgainVariant=Passthrough  TsampIntegralVariant=Disabled_SignalSpec  ExternalSaturationOutDataTypeStr=Inherit: Same as second input  DerivativeSourceVariant=Disabled  PreIntVariant=InternalPreInt
  draw_total : Sum
  eF : Sum  Inputs=+-
  inv_Fslack : Gain  Gain=1/F_slack
  mode_draw : Product
  one : Constant
  one_minus : Sum  Inputs=+-
  slack_sat : Saturate  UpperLimit=1  LowerLimit=0
  takeup_gain : Gain  Gain=draw_takeup
  w_ff : Product  Inputs=*/
  w_lim : Saturate  UpperLimit=w_max  LowerLimit=w_min
  w_ref : Sum
  omega_ref : Outport
  wires:
  vline/1 -> w_ff/1
  r/1 -> w_ff/2
  Fref/1 -> eF/1
  F/1 -> eF/2, inv_Fslack/1  "eF"
  eF/1 -> PI_F/1
  inv_Fslack/1 -> one_minus/2
  one/1 -> one_minus/1
  one_minus/1 -> slack_sat/1
  slack_sat/1 -> takeup_gain/1
  PI_F/1 -> draw_total/1
  takeup_gain/1 -> draw_total/2
  mode/1 -> mode_draw/1
  draw_total/1 -> mode_draw/2
  w_ff/1 -> w_ref/1
  mode_draw/1 -> w_ref/2
  w_ref/1 -> w_lim/1
  w_lim/1 -> omega_ref/1

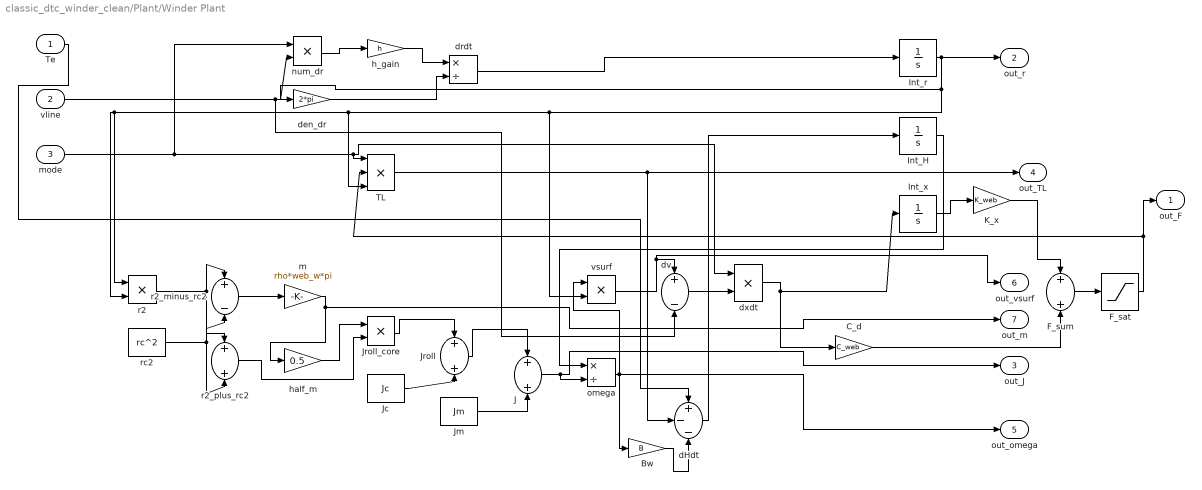
== system classic_dtc_winder_clean/Plant/Winder Plant ==
  Te : Inport
  vline : Inport  Port=2
  mode : Inport  Port=3
  Bw : Gain  Gain=B
  C_d : Gain  Gain=C_web
  F_sat : Saturate  UpperLimit=Fmax  LowerLimit=0
  F_sum : Sum
  Int_H : Integrator  InitialCondition=H0
  Int_r : Integrator  InitialCondition=r0  LimitOutput=on  UpperSaturationLimit=rmax  LowerSaturationLimit=rc
  Int_x : Integrator  InitialCondition=F0/K_web  LimitOutput=on  UpperSaturationLimit=Fmax/K_web  LowerSaturationLimit=0
  J : Sum
  Jc : Constant  Value=Jc
  Jm : Constant  Value=Jm
  Jroll : Sum
  Jroll_core : Product
  K_x : Gain  Gain=K_web
  TL : Product  Inputs=3
  dHdt : Sum  Inputs=+--
  den_dr : Gain  Gain=2*pi
  drdt : Product  Inputs=*/
  dv : Sum  Inputs=+-
  dxdt : Product
  h_gain : Gain  Gain=h
  half_m : Gain  Gain=0.5
  m : Gain  Gain=rho*web_w*pi
  num_dr : Product
  omega : Product  Inputs=*/
  r2 : Product
  r2_minus_rc2 : Sum  Inputs=+-
  r2_plus_rc2 : Sum
  rc2 : Constant  Value=rc^2
  vsurf : Product
  out_F : Outport
  out_r : Outport  Port=2
  out_J : Outport  Port=3
  out_TL : Outport  Port=4
  out_omega : Outport  Port=5
  out_vsurf : Outport  Port=6
  out_m : Outport  Port=7
  wires:
  Int_r/1 -> r2/1, r2/2, TL/3, vsurf/2, den_dr/1, out_r/1
  r2/1 -> r2_minus_rc2/1, r2_plus_rc2/1
  rc2/1 -> r2_minus_rc2/2, r2_plus_rc2/2
  r2_minus_rc2/1 -> m/1
  m/1 -> half_m/1, out_m/1
  half_m/1 -> Jroll_core/1
  r2_plus_rc2/1 -> Jroll_core/2
  Jroll_core/1 -> Jroll/1
  Jc/1 -> Jroll/2
  Jroll/1 -> J/1
  Jm/1 -> J/2
  Int_H/1 -> omega/1
  J/1 -> omega/2, out_J/1
  mode/1 -> TL/1, dxdt/1, num_dr/1
  F_sat/1 -> TL/2, out_F/1
  omega/1 -> vsurf/1, Bw/1, out_omega/1
  vline/1 -> num_dr/2, dv/2
  num_dr/1 -> h_gain/1
  h_gain/1 -> drdt/1
  den_dr/1 -> drdt/2
  Te/1 -> dHdt/1
  TL/1 -> dHdt/2, out_TL/1
  Bw/1 -> dHdt/3
  vsurf/1 -> dv/1, out_vsurf/1
  dv/1 -> dxdt/2
  drdt/1 -> Int_r/1
  dHdt/1 -> Int_H/1
  dxdt/1 -> Int_x/1, C_d/1
  Int_x/1 -> K_x/1
  K_x/1 -> F_sum/1
  C_d/1 -> F_sum/2
  F_sum/1 -> F_sat/1

== matlab function classic_dtc_winder_clean/Controller/MATLAB Function1 ==
  data: lambda_s_mag input; Sa output; theta_s_deg input; Te_est input; lambda_ref input; Te_ref input; HB_lambda input; HB_torque input; Sb output; Sc output
function [Sa, Sb, Sc] = dtc_switching_table(lambda_s_mag, theta_s_deg, Te_est, ...
    lambda_ref, Te_ref, HB_lambda, HB_torque)
%#codegen
% DTC hysteresis comparators + switching table (Parts 4.4-4.6)
% Outputs the 3-phase switching state (Sa,Sb,Sc) each in {0,1}
% Feed this into a Simulink "Controlled Voltage Source" / averaged VSI
% block, or directly into a full switched IGBT bridge if you're doing
% detailed power-electronics simulation.

persistent d_lambda d_torque
if isempty(d_lambda)
    d_lambda = 1;   % start assuming flux needs to rise
    d_torque = 0;
end

%% --- Flux hysteresis comparator (2-level, Part 4.4) ---
flux_err = lambda_ref - lambda_s_mag;
if flux_err > HB_lambda
    d_lambda = 1;
elseif flux_err < -HB_lambda
    d_lambda = 0;
end
% else: hold previous value (hysteresis behavior)

%% --- Torque hysteresis comparator (3-level, Part 4.4) ---
torque_err = Te_ref - Te_est;
if torque_err > HB_torque
    d_torque = 1;
elseif torque_err < -HB_torque
    d_torque = -1;
else
    d_torque = 0;
end

%% --- Sector identification (Step 1 from the sector clarification) ---
theta = mod(theta_s_deg, 360);
if theta >= 330 || theta < 30
    n = 1;
elseif theta < 90
    n = 2;
elseif theta < 150
    n = 3;
elseif theta < 210
    n = 4;
elseif theta < 270
    n = 5;
else
    n = 6;
end

%% --- Vector selection rule (Step 2 from the sector clarification) ---
% Vector index wraps mod 6, mapped to 1-6 (no zero index)
wrap6 = @(k) mod(k-1,6) + 1;

if d_torque == 0
    vec_idx = 0;   % zero vector (alternate V0/V7 for switching loss balance)
elseif d_lambda == 1 && d_torque == 1
    vec_idx = wrap6(n+1);
elseif d_lambda == 1 && d_torque == -1
    vec_idx = wrap6(n-1);
elseif d_lambda == 0 && d_torque == 1
    vec_idx = wrap6(n+2);
else % d_lambda == 0 && d_torque == -1
    vec_idx = wrap6(n-2);
end

%% --- Map vector index to switching state (Part 3.2 table) ---
switch vec_idx
    case 0
        Sa = 0; Sb = 0; Sc = 0;     % V0 (use V7=[1 1 1] on alternating cycles)
    case 1
        Sa = 1; Sb = 0; Sc = 0;     % V1
    case 2
        Sa = 1; Sb = 1; Sc = 0;     % V2
    case 3
        Sa = 0; Sb = 1; Sc = 0;     % V3
    case 4
        Sa = 0; Sb = 1; Sc = 1;     % V4
    case 5
        Sa = 0; Sb = 0; Sc = 1;     % V5
    case 6
        Sa = 1; Sb = 0; Sc = 1;     % V6
    otherwise
        % Should be unreachable given vec_idx is always 0-6, but
        % MATLAB Coder requires every output defined on every path.
        Sa = 0; Sb = 0; Sc = 0;
end

end

== matlab function classic_dtc_winder_clean/Controller/dtc_estimator ==
  settings: updateMethod=DISCRETE
  data: ia input; lambda_s_mag output; ib input; ic input; v_alpha input; v_beta input; Rs input; p input; Ts input; theta_s_deg output; Te_est output; lambda_alpha output; lambda_beta output; i_beta output
function [lambda_s_mag, theta_s_deg, Te_est, lambda_alpha, lambda_beta, i_beta] = dtc_estimator(ia, ib, ic, v_alpha, v_beta, Rs, p, Ts)
%#codegen
% DTC flux and torque estimator (voltage model, Part 4.3)
% Implements this as a MATLAB Function block with two persistent
% integrator states (lambda_alpha, lambda_beta).
%
% Inputs:
%   ia, ib, ic      - measured phase currents [A]
%   v_alpha, v_beta - inverter output voltage in alpha-beta frame [V]
%                     (computed upstream from the switching state, Part 3.2)
%   Rs              - stator resistance [ohm]
%   p               - pole pairs
%   Ts              - sample time [s]
%
% Outputs:
%   lambda_s_mag - stator flux magnitude [Wb]
%   theta_s_deg  - stator flux angle [deg], wrapped to [0,360)
%   Te_est       - estimated electromagnetic torque [N*m]
%   lambda_alpha, lambda_beta - flux components, useful for scope/debug

%{
This is the block that answers the two questions torque control actually depends on: how big is my stator flux, and what angle is it 
at relative to where it started — recall from Part 4.2, torque depends on the angle between stator flux and rotor flux, 
and this angle is embedded in how theta_s_deg evolves over time.
%}


persistent lam_a lam_b
if isempty(lam_a)
    lam_a = 0.175;
    lam_b = 0;
end
%% Correct physical current inversion from the sensors
ia_true = -ia;
ib_true = -ib;

%% Clarke transform of true currents
i_alpha = ia_true;
i_beta  = (1/sqrt(3))*ia_true + (2/sqrt(3))*ib_true;

%% Flux integration (Part 4.3) — forward Euler, simplest form
% NOTE: pure integration drifts at low speed (Problem 3, Part 5.1).
% Once this base version works, replace with a low-pass-filter-based
% or closed-loop observer estimator and compare.
lam_a = lam_a + Ts * (v_alpha - Rs*i_alpha);
lam_b = lam_b + Ts * (v_beta  - Rs*i_beta);


lambda_alpha = lam_a;
lambda_beta  = lam_b;

%% Magnitude and angle
lambda_s_mag = sqrt(lam_a^2 + lam_b^2);
theta_s_rad  = atan2(lam_b, lam_a);
theta_s_deg  = mod(theta_s_rad * 180/pi, 360);

%% Torque estimate (Part 4.3)
Te_est = 1.5 * p * (lam_a*i_beta - lam_b*i_alpha);

end

== matlab function classic_dtc_winder_clean/Controller/MATLAB Function ==
  data: Sa input; v_alpha output; Sb input; Sc input; Vdc input; v_beta output
function [v_alpha, v_beta] = calculate_voltages(Sa, Sb, Sc, Vdc)
% Calculate alpha-beta voltages based on switching states and DC link
v_alpha = (2/3) * Vdc * (Sa - 0.5 * (Sb + Sc));
v_beta  = (2/3) * Vdc * (sqrt(3)/2) * (Sb - Sc);
end

%{
Inputs: Sa, Sb, Sc (the switching state chosen last cycle), Vdc
Outputs: v_alpha, v_beta

This answers: given the switch positions I already commanded, what voltage is actually sitting on the motor terminals right now? 
It doesn't measure anything — it's a pure calculation from Part 3.2's formula, because a 2-level inverter's output voltage is fully determined by which switches are on. 
This is one of the things that makes DTC elegant: you never need a voltage sensor, just knowledge of your own last command plus Vdc.

This feeds straight into the estimator, because the estimator needs to know "how much voltage pushed the flux where it is now."
%}
